simulink model "injector_component_test"  (R2026a)
settings: Solver=VariableStepAuto  StopTime=1
libraries: fl_lib x4, nesl_utility x2, SimscapeFluids_lib x1
settings Model: Creator=giuse  LastModifiedBy=giuse

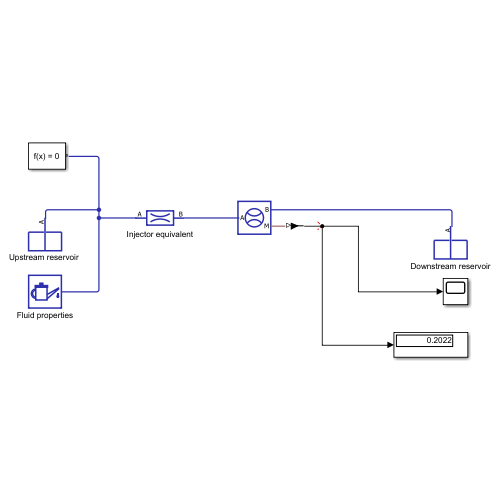
[thumbnail: Simulink's stored preview of the top-level diagram]
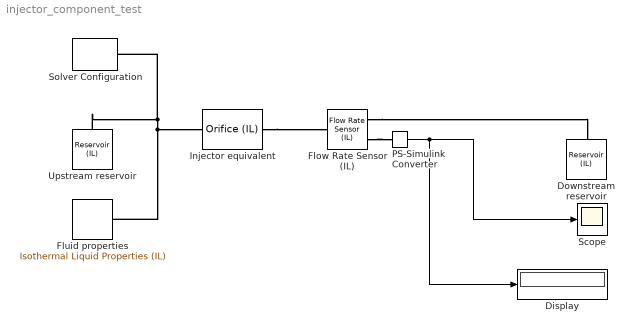
== system injector_component_test ==
  Display : Display
  Downstream reservoir : fl_lib/Isothermal Liquid/Elements/Reservoir (IL)  pressure_input=false  pressure_spec=foundation.enum.pressure_spec.specified  reservoir_pressure=0.5 MPa
  Flow Rate Sensor (IL) : fl_lib/Isothermal Liquid/Sensors/Flow Rate Sensor (IL)  sensor_type=foundation.enum.mass_volumetric_sensor.mass
  Fluid properties : fl_lib/Isothermal Liquid/Utilities/Isothermal Liquid Properties (IL)  rho_L_atm=998.21 kg/m^3  bulk_modulus_model=foundation.enum.bulk_modulus_model.const  beta_gain=6  beta_L_atm=2.1791e9 Pa  nu_atm=1.0034e-6 m^2/s  p_atm=0.101325 MPa  p_min=1 Pa  properties_range_check=simscape.enum.assert.action.error  air_fraction=0  polytropic_index=1.0  rho_g_atm=1.225 kg/m^3  air_dissolution_model=false  p_crit=3 MPa
  Injector equivalent : SimscapeFluids_lib/Isothermal Liquid/Valves & Orifices/Orifices/Orifice (IL)  orifice_type=foundation.enum.constant_variable.constant  constant_orifice_spec=fluids.isothermal_liquid.valves_orifices.orifices.enum.constant_orifice_spec.area  variable_orifice_spec=fluids.isothermal_liquid.valves_orifices.orifices.enum.orifice_spec.linear  orifice_area_constant=1e-5 m^2  p_diff_TLU_constant=[-4, -3, -2, -1, -.5, 0, .5, 1, 2, 3, 4] MPa  vol_flow_TLU_constant=[-2.44, -2.12, -1.68, -1.22, -.84, 0, .85, 1.21, 1.7, 2.09, 2.41] .* 1e-3 m^3/s  S_min=0 m  del_S=5e-3 m  open_orientation=fluids.isothermal_liquid.valves_orifices.orifices.enum.orifice_orientation.positive  area_max=1e-4 m^2  area_leak=1e-10 m^2  S_TLU=[0, .002, .004, .007, .017] m  orifice_area_TLU=[1e-09, 2.0352e-07, 4.0736e-05, .00011438, .00034356] m^2  area=inf m^2  Cd=0.64  Re_c=150  smoothing_factor=0.01  pressure_recovery=false  S_vol_flow_TLU=[0, .002, .004, .007, .017] m  p_diff_TLU=[.3, .5, .7] MPa  vol_flow_TLU=1e-3 * [1.7e-05, 2e-05, 2.6e-05; .0035, .0045, .0053; .7, .9, 1.06; 1.96, 2.5, 3; 6, 7.7, 9.13] m^3/s
  PS-Simulink Converter : nesl_utility/PS-Simulink Converter  PhysicalDomain=network_engine_domain  SubClassName=ps_output  LeftPortType=input  RightPortType=output  PseudoPeriodic=off  Frequencies=[]  VectorFormat=inherit  Unit=kg/s  AffineConversion=off
  Scope : Scope
      settings: ActiveDisplayYMinimum=0.13391864516247554  ActiveDisplayYMaximum=0.283161724489801
  Solver Configuration : nesl_utility/Solver Configuration  PhysicalDomain=network_engine_domain  SubClassName=solver  LeftPortType=input  RightPortType=generic  Tones=[]  Harmonics=[]  SimulateNoise=off  Profile=off  UseLocalSampling=off  EnableSwitchedLinearOptims=on  FrequencyDomain=off  UseCCode=off  RelTol=0.001  AbsTol=0.001  MinStep=1e-09  ToWorkspace=off  RevertToSquareIcSolve=off  NumHomotopyIterations=100  PhasorMode=off  PhasorModeNumHarmonics=1  ConsistencySolver=NEWTON_XTOL_AFTER_FTOL  CanonicalOrdering=CANONICAL  OptimizeIntermediates=OPTIMIZED  IndexReductionMethod=DerivativeReplacement  DoDC=off  ResidualTolerance=1e-09  ConsistencyTolSource=GLOBAL  ConsistencyAbsTol=0.001  ConsistencyRelTol=0.001  ConsistencyTolFactor=0.001  UseLocalSolver=off  LocalSolverChoice=NE_BACKWARD_EULER_ADVANCER  ResolveIndetEquations=on  FunctionEvalNumThread=1  LocalSolverSampleTime=0.001  DoFixedCost=off  MaxNonlinIter=3  MaxModeIter=2  ComputeImpulses=off  ImpulseIterations=2  LinearAlgebra=auto  LinearAlgebraNumThread=0  EquationFormulation=NE_TIME_EF  DelaysMemoryBudget=1024  AutomaticFiltering=on  FilteringTimeConstant=0.001  PartitionStorageMethod=AS_NEEDED  PartitionMemoryBudget=1024  PartitionMethod=ROBUST  MultibodyUseLocalSolver=off  MultibodyLocalSolverChoice=ODE1  MultibodyLocalSolverSampleTime=0.001
  "Upstream reservoir " : fl_lib/Isothermal Liquid/Elements/Reservoir (IL)  pressure_input=false  pressure_spec=foundation.enum.pressure_spec.specified  reservoir_pressure=1 MPa
  wires:
  PS-Simulink Converter/1 -> Display/1, Scope/1
  connections:
  "Upstream reservoir "/LConn1 -- Fluid properties/RConn1 -- Injector equivalent/LConn1 -- Solver Configuration/RConn1
  Injector equivalent/RConn1 -- Flow Rate Sensor (IL)/LConn1
  Flow Rate Sensor (IL)/RConn1 -- Downstream reservoir/LConn1
  Flow Rate Sensor (IL)/RConn2 -- PS-Simulink Converter/LConn1
